simulink model "TS_IOTcommunication"  (R2025b)
settings: Solver=FixedStepAuto  StartTime=0.0  StopTime=inf  RelTol=1e-3  EnableMultiTasking=on
libraries: raspberrypiIOTlib x2, simulink x1
settings Model: ExtModeTrigDuration=2  Creator=sport  LastModifiedBy=sport
settings SolverCC: PositivePriorityOrder=on
settings OptimizationCC: EnhancedBackFolding=on  PassReuseOutputArgsAs=Individual arguments  ZeroExternalMemoryAtStartup=off  ZeroInternalMemoryAtStartup=off  MaxStackSize=200000  OptimizeBlockOrder=speed  DifferentSizesBufferReuse=on  OptimizationCustomize=off  EfficientTunableParamExpr=on
settings DebuggingCC: ParameterTunabilityLossMsg=error
settings HardwareCC: ProdBitPerPointer=32.0  ProdBitPerSizeT=32.0  ProdBitPerPtrDiffT=32.0  ProdLargestAtomicInteger=Long  ProdLargestAtomicFloat=Double  ProdWordSize=32.0  ProdLongLongMode=on  ProdHWDeviceType=ARM Compatible->ARM Cortex-A (32-bit)
settings RTWCC: SystemTargetFile=ert.tlc  HardwareBoard=Raspberry Pi  TLCOptions="-aInlineSetEventsForThisBaseRateFcn=TLC_FALSE -aSuppressMultiTaskScheduler=TLC_FALSE  -aRateBasedStepFcn=0"  TemplateMakefile=ert_default_tmf  Toolchain=GNU GCC Embedded Linux  BuildConfiguration=Faster Runs  Description=Embedded Coder
settings CodeAppCC: ForceParamTrailComments=on  IgnoreCustomStorageClasses=off  OperatorAnnotations=on  SimulinkDataObjDesc=on  SFDataObjDesc=on  InsertBlockDesc=on
settings ERTTargetCC: ExtModeTransport=2.0  ExtModeStaticAlloc=on  ExtModeMexFile=ext_xcp  ExtModeIntrfLevel=Level2 - Open  InlinedParameterPlacement=Hierarchical  CodeReplacementLibrary=ARM Cortex-A CMSIS  SupportVariableSizeSignals=on

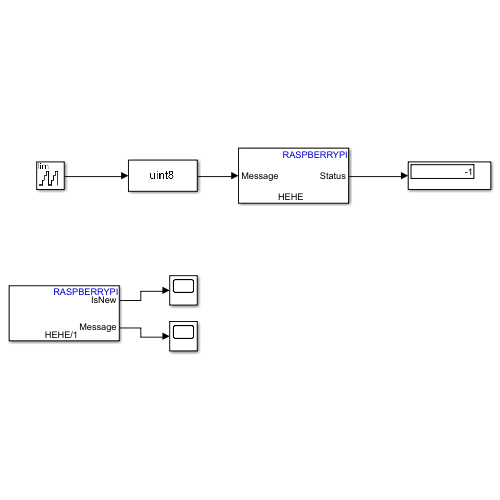
[thumbnail: Simulink's stored preview of the top-level diagram]
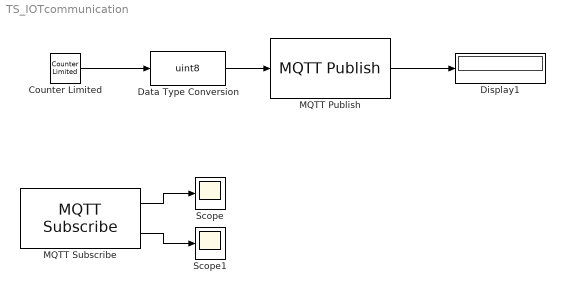
== system TS_IOTcommunication ==
  Counter Limited : simulink/Sources/Counter Limited  uplimit=1000  tsamp=1
  Data Type Conversion : DataTypeConversion  OutDataTypeStr=uint8  SaturateOnIntegerOverflow=off  RndMeth=Floor
  Display1 : Display
  MQTT Publish : raspberrypiIOTlib/MQTT Publish  Topic=HEHE  QoS=0  RetainMsg=off  blockPlatform=RASPBERRYPI
  MQTT Subscribe : raspberrypiIOTlib/MQTT Subscribe  Topic=HEHE/1  QoS=0  MessageLength=1  OutputMessage=off  SampleTime=1  blockPlatform=RASPBERRYPI
  Scope : Scope
      settings: ActiveDisplayYMinimum=-146.15641682769569  ActiveDisplayYMaximum=106.33684487413917
  Scope1 : Scope
      settings: ActiveDisplayYMinimum=-55.419042711405382  ActiveDisplayYMaximum=46.687544348208291
  wires:
  Counter Limited/1 -> Data Type Conversion/1
  Data Type Conversion/1 -> MQTT Publish/1
  MQTT Publish/1 -> Display1/1
  MQTT Subscribe/2 -> Scope1/1
  MQTT Subscribe/1 -> Scope/1
